simulink model "RLS_LIT"  (R2024a)
settings: Solver=FixedStepAuto  StartTime=0.0  StopTime=0.6  FixedStep=10e-6  RelTol=1e-3
settings Model: PacingRate=1.300000  Creator=Raphael Teixeira  LastModifiedBy=Raphael Teixeira

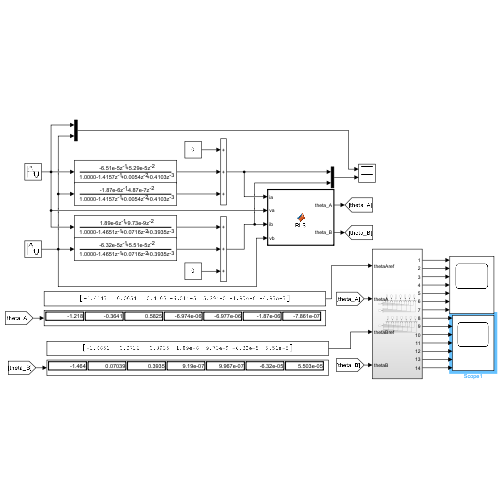
[thumbnail: Simulink's stored preview of the top-level diagram]
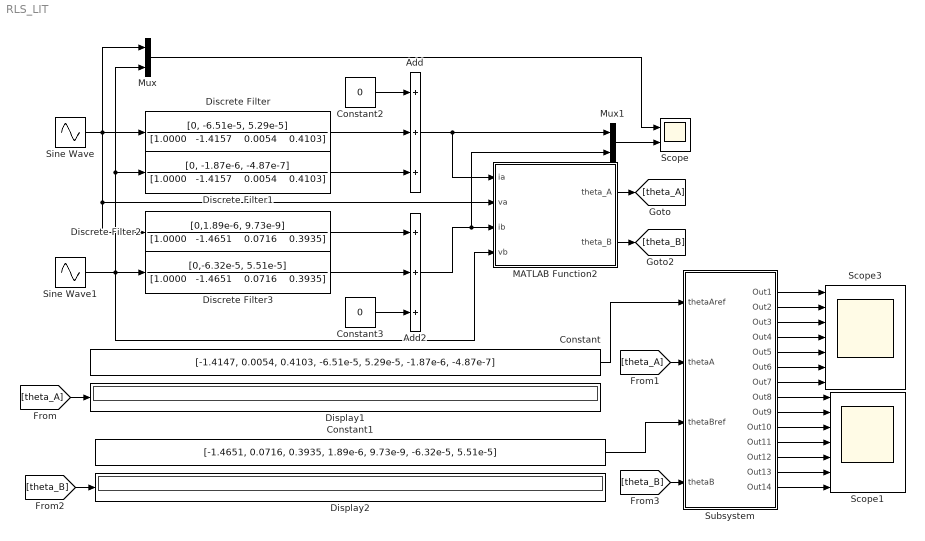
== system RLS_LIT ==
  Add : Sum  Inputs=+++
  Add2 : Sum  Inputs=+++
  Constant : Constant  Value=[-1.4147, 0.0054, 0.4103, -6.51e-5, 5.29e-5, -1.87e-6, -4.87e-7]  SampleTime=10e-6
  Constant1 : Constant  Value=[-1.4651, 0.0716, 0.3935, 1.89e-6, 9.73e-9, -6.32e-5, 5.51e-5]  SampleTime=10e-6
  Constant2 : Constant  Value=0
  Constant3 : Constant  Value=0
  Discrete Filter : DiscreteFilter  Numerator=[0, -6.51e-5, 5.29e-5]  Denominator="[1.0000   -1.4157    0.0054    0.4103]"
  Discrete Filter1 : DiscreteFilter  Numerator=[0, -1.87e-6, -4.87e-7]  Denominator="[1.0000   -1.4157    0.0054    0.4103]"
  Discrete Filter2 : DiscreteFilter  Numerator=[0,1.89e-6, 9.73e-9]  Denominator="[1.0000   -1.4651    0.0716    0.3935]"
  Discrete Filter3 : DiscreteFilter  Numerator=[0,-6.32e-5, 5.51e-5]  Denominator="[1.0000   -1.4651    0.0716    0.3935]"
  Display1 : Display
  Display2 : Display
  MATLAB Function2 : MATLAB Function  TreatAsAtomicUnit=on
  Mux : Mux  Inputs=2
  Mux1 : Mux  Inputs=2
  Scope : Scope  NumInputPorts=2
  Scope1 : Scope  NumInputPorts=7
  Scope3 : Scope  NumInputPorts=7
  Sine Wave : Sin  Amplitude=110  Frequency=60  SampleTime=10e-6
  Sine Wave1 : Sin  Amplitude=110  Frequency=60  Phase=-pi/2  SampleTime=10e-6
  Subsystem : Subsystem
  wires:
  Add/1 -> Mux1/1, MATLAB Function2/1(ia)
  Discrete Filter3/1 -> Add2/2
  Discrete Filter2/1 -> Add2/1
  Discrete Filter/1 -> Add/2
  Discrete Filter1/1 -> Add/3
  Constant2/1 -> Add/1
  Add2/1 -> Mux1/2, MATLAB Function2/3(ib)
  MATLAB Function2/1(theta_A) -> [theta_A]
  MATLAB Function2/2(theta_B) -> [theta_B]
  [theta_B] -> Display2/1
  [theta_A] -> Display1/1
  Subsystem/1(Out1) -> Scope3/1
  Subsystem/2(Out2) -> Scope3/2
  Subsystem/3(Out3) -> Scope3/3
  Subsystem/4(Out4) -> Scope3/4
  Subsystem/5(Out5) -> Scope3/5
  Subsystem/6(Out6) -> Scope3/6
  Subsystem/7(Out7) -> Scope3/7
  Subsystem/8(Out8) -> Scope1/1
  Subsystem/9(Out9) -> Scope1/2
  Subsystem/10(Out10) -> Scope1/3
  Subsystem/11(Out11) -> Scope1/4
  Subsystem/12(Out12) -> Scope1/5
  Subsystem/13(Out13) -> Scope1/6
  Subsystem/14(Out14) -> Scope1/7
  Constant/1 -> Subsystem/1(thetaAref)
  [theta_A] -> Subsystem/2(thetaA)
  [theta_B] -> Subsystem/4(thetaB)
  Constant1/1 -> Subsystem/3(thetaBref)
  Constant3/1 -> Add2/3
  Mux/1 -> Scope/1
  Mux1/1 -> Scope/2
  Sine Wave1/1 -> MATLAB Function2/4(vb), Mux/2, Discrete Filter1/1, Discrete Filter3/1
  Sine Wave/1 -> Mux/1, MATLAB Function2/2(va), Discrete Filter2/1, Discrete Filter/1

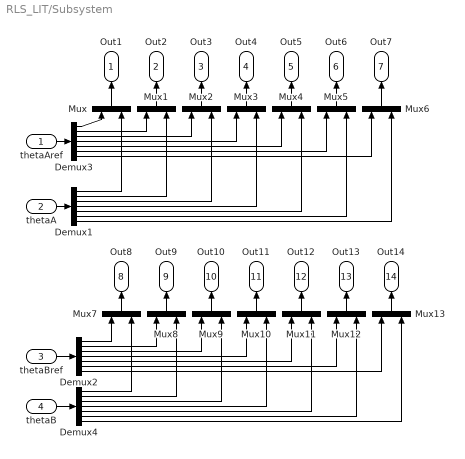
== system RLS_LIT/Subsystem ==
  thetaAref : Inport
  thetaA : Inport  Port=2
  thetaBref : Inport  Port=3
  thetaB : Inport  Port=4
  Demux{1..4} (4 alike) : Demux  Outputs=7
  Mux{,1..13} (14 alike) : Mux  Inputs=2
  Out1 : Outport
  Out2 : Outport  Port=2
  Out3 : Outport  Port=3
  Out4 : Outport  Port=4
  Out5 : Outport  Port=5
  Out6 : Outport  Port=6
  Out7 : Outport  Port=7
  Out8 : Outport  Port=8
  Out9 : Outport  Port=9
  Out10 : Outport  Port=10
  Out11 : Outport  Port=11
  Out12 : Outport  Port=12
  Out13 : Outport  Port=13
  Out14 : Outport  Port=14
  wires:
  Demux1/1 -> Mux/2
  Demux2/2 -> Mux8/1
  Demux1/3 -> Mux2/2
  Demux1/7 -> Mux6/2
  Demux1/2 -> Mux1/2
  Demux1/6 -> Mux5/2
  Demux1/4 -> Mux3/2
  Demux1/5 -> Mux4/2
  thetaAref/1 -> Demux3/1
  Demux3/1 -> Mux/1
  Demux3/2 -> Mux1/1
  Demux3/3 -> Mux2/1
  Demux3/4 -> Mux3/1
  Demux3/5 -> Mux4/1
  Demux3/6 -> Mux5/1
  Demux3/7 -> Mux6/1
  Mux/1 -> Out1/1
  Mux1/1 -> Out2/1
  Mux2/1 -> Out3/1
  Mux3/1 -> Out4/1
  Mux4/1 -> Out5/1
  Mux5/1 -> Out6/1
  Mux6/1 -> Out7/1
  thetaA/1 -> Demux1/1
  thetaBref/1 -> Demux2/1
  thetaB/1 -> Demux4/1
  Mux13/1 -> Out14/1
  Mux12/1 -> Out13/1
  Mux11/1 -> Out12/1
  Mux10/1 -> Out11/1
  Mux9/1 -> Out10/1
  Mux8/1 -> Out9/1
  Mux7/1 -> Out8/1
  Demux2/1 -> Mux7/1
  Demux4/1 -> Mux7/2
  Demux4/2 -> Mux8/2
  Demux2/3 -> Mux9/1
  Demux2/4 -> Mux10/1
  Demux2/5 -> Mux11/1
  Demux2/6 -> Mux12/1
  Demux2/7 -> Mux13/1
  Demux4/3 -> Mux9/2
  Demux4/4 -> Mux10/2
  Demux4/5 -> Mux11/2
  Demux4/6 -> Mux12/2
  Demux4/7 -> Mux13/2

== matlab function RLS_LIT/MATLAB Function2 ==
  data: theta_A output; ia input; va input; ib input; theta_B output; vb input
function [theta_A, theta_B] = RLS(ia, va, ib, vb)

    % Declara parâmetros ajustáveis como persistentes:
    persistent Pa Pb Ia Ib Va Vb Ka Kb lambda
    persistent theta_a theta_b

    % Inicializa parâmetros do RLS:
    if isempty(Pa)
        nA = 3;
        nB = 2;
        nparams = nA + 2*nB;
        Pa =  1e8*eye(nparams);
        Pb =  1e8*eye(nparams);
        lambda = 0.99;
        theta_a = zeros(nparams,1);
        theta_b = zeros(nparams,1);
        Ia = zeros(1,nA+1);
        Ib = zeros(1,nA+1);
        Va = zeros(1,nB+1);
        Vb = zeros(1,nB+1);
    end
    
    % Vetor de amostras das variáveis:
    Ia = [ia, Ia(1,1:end-1)];
    Ib = [ib, Ib(1,1:end-1)];
    Va = [va, Va(1,1:end-1)];
    Vb = [vb, Vb(1,1:end-1)];

    % Vetor de regressão 
    phi_a = [-Ia(1,2:end), Va(1,2:end), Vb(1,2:end)]';
    phi_b = [-Ib(1,2:end), Va(1,2:end), Vb(1,2:end)]';

    % Atualização do RLS para eixo alpha
    Ka = Pa*phi_a / (lambda + phi_a' * Pa * phi_a);
    theta_a = theta_a + Ka*(ia - phi_a'*theta_a);
    Pa = (Pa - Ka * phi_a' * Pa) / lambda;

    % Atualização do RLS para eixo alpha
    Kb = Pb * phi_b / (lambda + phi_b' * Pb * phi_b);
    theta_b = theta_b + Kb*(ib - phi_b'*theta_b);
    Pb = (Pb - Kb * phi_b' * Pb) / lambda;

    theta_A = theta_a;
    theta_B = theta_b;

end
